simulink model "CLVF"  (R2020a)
settings: Solver=FixedStepAuto  StartTime=0.0  StopTime=tsim  FixedStep=baseRate  RelTol=1e-3  EnableMultiTasking=on
values from neighbouring files (symbols this model uses):
  a = sqrt(sum(aTimesOVec.^2))    [Run_Initializer.m]    (also in a_max_CLVF2D.m = params(4))
  a_max = 0.4/BLACKMass    [Run_Initializer.m]
  a_prime = newParams(2)    [Run_Initializer.m]    (also in a_max_LVF.m = params(2))
  acceptableRadius = 0.05    [Run_Initializer.m]
  b = newParams(3)    [Run_Initializer.m]    (also in a_max_CLVF2D.m = params(3))
  baseRate = 0.05    [Run_Initializer.m]
  BLACKMass = model_param(3)    [Run_Initializer.m]
  d = [0.16;0.542;0]    [Run_Initializer.m]    (also in a_max_LVF.m = [rotStuff(3);rotStuff(4);rotStuff(5)])
  drop_states_BLACK = rC_I0    [Run_Initializer.m]
  drop_states_BLUE = [ xLength/2+0.9; yLength/2+0.5; 0]    [Run_Initializer.m]
  drop_states_RED = rT_I0    [Run_Initializer.m]
  F_thrusters_BLACK = 0.25.*ones(8,1)    [Run_Initializer.m]
  F_thrusters_BLUE = 0.25.*ones(8,1)    [Run_Initializer.m]
  F_thrusters_RED = 0.25.*ones(8,1)    [Run_Initializer.m]
  home_states_BLACK = [ xLength/2+0.4; yLength/2; 0]    [Run_Initializer.m]
  home_states_BLUE = [ xLength/2-0.9; yLength/2+0.5; 0]    [Run_Initializer.m]
  home_states_RED = [ xLength/2-0.4; yLength/2; 0]    [Run_Initializer.m]
  init_states_BLACK = rC_I0    [Run_Initializer.m]
  init_states_BLUE = [ xLength/2+0.9; yLength/2+0.5; 0]    [Run_Initializer.m]
  init_states_RED = rT_I0    [Run_Initializer.m]
  k_v_rel = 2*v_max/a_prime    (= 1)    [Run_Initializer.m]
  ka = newParams(2)    [Run_Initializer.m]    (also in a_max_CLVF2D.m = params(2))
  kc = newParams(1)    [Run_Initializer.m]    (also in a_max_CLVF2D.m = params(1))
  kd = 5.0    (= 5)    [Run_Initializer.m]
  Kd_tb = 0.4    [Run_Initializer.m]
  Kd_tblue = 0.4    [Run_Initializer.m]
  Kd_tr = 0.4    [Run_Initializer.m]
  Kd_xb = 5    [Run_Initializer.m]
  Kd_xblue = 5    [Run_Initializer.m]
  Kd_xr = 5    [Run_Initializer.m]
  Kd_yb = 5    [Run_Initializer.m]
  Kd_yblue = 5    [Run_Initializer.m]
  Kd_yr = 5    [Run_Initializer.m]
  Kp_tb = 0.1    [Run_Initializer.m]
  Kp_tblue = 0.1    [Run_Initializer.m]
  Kp_tr = 0.1    [Run_Initializer.m]
  Kp_xb = 2    [Run_Initializer.m]
  Kp_xblue = 2    [Run_Initializer.m]
  Kp_xr = 2    [Run_Initializer.m]
  Kp_yb = 2    [Run_Initializer.m]
  Kp_yblue = 2    [Run_Initializer.m]
  Kp_yr = 2    [Run_Initializer.m]
  noise_variance_BLACK = 0    [Run_Initializer.m]
  noise_variance_BLUE = 0    [Run_Initializer.m]
  noise_variance_RED = 0    [Run_Initializer.m]
  o_hat_B = aTimesOVec./a    [Run_Initializer.m]
  o_hat_prime = o_prime/sqrt(sum(o_prime.^2))    [Run_Initializer.m]
  Phase0_End = Phase0_Duration    (= 10)    [Run_Initializer.m]
  Phase1_End = Phase0_Duration + Phase1_Duration    (= 15)    [Run_Initializer.m]
  Phase2_End = Phase0_Duration + Phase1_Duration +                                   Phase2_Duration    (= 35)    [Run_Initializer.m]
  Phase3_End = Phase0_Duration + Phase1_Duration +                                   Phase2_Duration + Phase3_Duration    [Run_Initializer.m]
  Phase3_SubPhase1_End = Phase2_End + Phase3_SubPhase1_Duration    (= 40)    [Run_Initializer.m]
  Phase3_SubPhase2_End = Phase2_End + Phase3_SubPhase1_Duration +                                   Phase3_SubPhase2_Duration    (= 45)    [Run_Initializer.m]
  Phase3_SubPhase3_End_BLACK = Phase2_End + Phase3_SubPhase1_Duration +                                   Phase3_SubPhase2_Duration +                                  Phase3_SubPhase3_Duration + Phase3_SubPhase3_and_a_half    (= 51)    [Run_Initializer.m]
  Phase3_SubPhase3_End_RED = Phase2_End + Phase3_SubPhase1_Duration +                                   Phase3_SubPhase2_Duration +                                  Phase3_SubPhase3_Duration    (= 46)    [Run_Initializer.m]
  Phase3_SubPhase4_End = Phase2_End + Phase3_SubPhase1_Duration +                                   Phase3_SubPhase2_Duration +                                  Phase3_SubPhase3_Duration +                                  Phase3_SubPhase4_Duration + Phase3_SubPhase3_and_a_half    [Run_Initializer.m]
  Phase4_End = Phase0_Duration + Phase1_Duration +                                   Phase2_Duration + Phase3_Duration +                                   Phase4_Duration    [Run_Initializer.m]
  Phase5_End = Phase0_Duration + Phase1_Duration +                                   Phase2_Duration + Phase3_Duration +                                   Phase4_Duration + Phase5_Duration    [Run_Initializer.m]
  r_co = r_co_over_a_prime*a_prime    (= 0.16)    [Run_Initializer.m]
  rC_I0 = [0.9*xLength;yLength/2-0.5;pi/2]    [Run_Initializer.m]
  rT_I0 = [yLength/2;yLength/2;possibleStarts(startingRotation)]    [Run_Initializer.m]
  serverRate = 0.1    [Run_Initializer.m]
  sys_BLACK = c2d(sys_BLACK_CONT, baseRate)    [Run_Initializer.m]
  sys_BLACK_ROT = c2d(sys_BLACK_rot_CONT, baseRate)    [Run_Initializer.m]
  sys_RED = c2d(sys_RED_CONT, baseRate)    [Run_Initializer.m]
  sys_RED_ROT = c2d(sys_RED_rot_CONT, baseRate)    [Run_Initializer.m]
  theta_d = 30*d2r    (= 0.523598775598)    [Run_Initializer.m]    (also in a_max_LVF.m = rotStuff(2))
  thruster_dist2CG_BLACK = [83.42;-52.58;55.94;-60.05;54.08;-53.92;77.06;-55.94]    [Run_Initializer.m]
  thruster_dist2CG_BLUE = [83.42;-52.58;55.94;-60.05;54.08;-53.92;77.06;-55.94]    [Run_Initializer.m]
  thruster_dist2CG_RED = [49.92;-78.08;70.46;-63.54;81.08;-50.42;57.44;-75.96]    [Run_Initializer.m]
  w_body = 6.0 * d2r    (= 0.10471975512)    [Run_Initializer.m]
undefined symbols (not defined in the file or in its folder): DiscIntNeverNeededParam, Discrete, Phase3_SubPhase3_End, platformSelection, simMode, Time, WhoAmI
libraries: dspstat3 x18, dspsigops x14, raspberrypiBasiclib x10, embdlinuxlib x8, simulink x8, ctrlSharedLib x4, mspfiltlib x3, dsparch4 x3, dspswit3 x2, MainLibrary x2, sensehatlib x1
(part 8 of 10)

== system CLVF/Gyroscope & Acceleration Algorithms/Change BLUE Behavior/Fix Initial Bias (Accel)/Correct AccelY/Calculate Running Mean ==
  In1 : Inport
  Action Port : ActionPort
  Delay : Delay  DelayLength=1
  Delay1 : Delay
  Delay2 : Delay  DelayLength=4
  Delay3 : Delay  DelayLength=5
  Delay4 : Delay  DelayLength=3
  Mean : dspstat3/Mean  run=off  InputProcessing=Columns as channels (frame based)  reset_popup=None  directionMode=Each column  dimension=1  roiEnable=off  roiType=Rectangles  roiPortion=Entire ROI  roiOutput=Individual statistics for each ROI  roiFlag=off  roundingMode=Floor  overflowMode=off  outputDataTypeStr=Inherit: Same as accumulator  outputMin=[]  outputMax=[]  outputLastDataTypeStr=Inherit: Same as accumulator
  Mux : Mux  Inputs=6
  Out1 : Outport
  wires:
  Delay3/1 -> Mux/6
  Delay2/1 -> Mux/5
  Delay1/1 -> Mux/3
  Delay4/1 -> Mux/4
  Delay/1 -> Mux/2
  In1/1 -> Delay3/1, Delay2/1, Delay4/1, Delay1/1, Delay/1, Mux/1
  Mux/1 -> Mean/1
  Mean/1 -> Out1/1

== system CLVF/Gyroscope & Acceleration Algorithms/Change BLUE Behavior/Fix Initial Bias (Accel)/Correct AccelY/Pass Current Accel ==
  In1 : Inport
  Action Port : ActionPort
  Out1 : Outport
  wires:
  In1/1 -> Out1/1

== system CLVF/Gyroscope & Acceleration Algorithms/Change BLUE Behavior/Fix Initial Bias (Accel)/Correct AccelY/Subsystem ==
  Universal_Time : DataStoreRead  DataStoreName=Univ_Time
  Time : Outport  VectorParamsAs1DForOutWhenUnconnected=off
  wires:
  Universal_Time/1 -> Time/1

== system CLVF/Gyroscope & Acceleration Algorithms/Change BLUE Behavior/Fix Initial Bias (Accel)/Correct AccelZ/Calculate Running Mean ==
  In1 : Inport
  Action Port : ActionPort
  Constant : Constant  Value=9.81
  Delay : Delay  DelayLength=1
  Delay1 : Delay
  Delay2 : Delay  DelayLength=4
  Delay3 : Delay  DelayLength=5
  Delay4 : Delay  DelayLength=3
  Mean : dspstat3/Mean  run=off  InputProcessing=Columns as channels (frame based)  reset_popup=None  directionMode=Each column  dimension=1  roiEnable=off  roiType=Rectangles  roiPortion=Entire ROI  roiOutput=Individual statistics for each ROI  roiFlag=off  roundingMode=Floor  overflowMode=off  outputDataTypeStr=Inherit: Same as accumulator  outputMin=[]  outputMax=[]  outputLastDataTypeStr=Inherit: Same as accumulator
  Mux : Mux  Inputs=6
  Subtract : Sum  Inputs=+-
  Out1 : Outport
  wires:
  Delay3/1 -> Mux/6
  Delay2/1 -> Mux/5
  Delay1/1 -> Mux/3
  Delay4/1 -> Mux/4
  Delay/1 -> Mux/2
  In1/1 -> Delay3/1, Delay2/1, Delay4/1, Delay1/1, Delay/1, Mux/1
  Mux/1 -> Mean/1
  Subtract/1 -> Out1/1
  Mean/1 -> Subtract/1
  Constant/1 -> Subtract/2

== system CLVF/Gyroscope & Acceleration Algorithms/Change BLUE Behavior/Fix Initial Bias (Accel)/Correct AccelZ/Pass Current Accel ==
  In1 : Inport
  Action Port : ActionPort
  Out1 : Outport
  wires:
  In1/1 -> Out1/1

== system CLVF/Gyroscope & Acceleration Algorithms/Change BLUE Behavior/Fix Initial Bias (Accel)/Correct AccelZ/Subsystem ==
  Universal_Time : DataStoreRead  DataStoreName=Univ_Time
  Time : Outport  VectorParamsAs1DForOutWhenUnconnected=off
  wires:
  Universal_Time/1 -> Time/1

== system CLVF/Gyroscope & Acceleration Algorithms/Change RED Behavior/Fix Initial Bias/Correct GyroX/Calculate Running Mean ==
  In1 : Inport
  Action Port : ActionPort
  Delay : Delay  DelayLength=1
  Delay1 : Delay
  Delay2 : Delay  DelayLength=4
  Delay3 : Delay  DelayLength=5
  Delay4 : Delay  DelayLength=3
  Mean : dspstat3/Mean  run=off  InputProcessing=Columns as channels (frame based)  reset_popup=None  directionMode=Each column  dimension=1  roiEnable=off  roiType=Rectangles  roiPortion=Entire ROI  roiOutput=Individual statistics for each ROI  roiFlag=off  roundingMode=Floor  overflowMode=off  outputDataTypeStr=Inherit: Same as accumulator  outputMin=[]  outputMax=[]  outputLastDataTypeStr=Inherit: Same as accumulator
  Mux : Mux  Inputs=6
  Out1 : Outport
  wires:
  Delay3/1 -> Mux/6
  Delay2/1 -> Mux/5
  Delay1/1 -> Mux/3
  Delay4/1 -> Mux/4
  Delay/1 -> Mux/2
  In1/1 -> Delay3/1, Delay2/1, Delay4/1, Delay1/1, Delay/1, Mux/1
  Mux/1 -> Mean/1
  Mean/1 -> Out1/1

== system CLVF/Gyroscope & Acceleration Algorithms/Change RED Behavior/Fix Initial Bias/Correct GyroX/Pass Current Gyro ==
  In1 : Inport
  Action Port : ActionPort
  Out1 : Outport
  wires:
  In1/1 -> Out1/1

== system CLVF/Gyroscope & Acceleration Algorithms/Change RED Behavior/Fix Initial Bias/Correct GyroX/Subsystem ==
  Universal_Time : DataStoreRead  DataStoreName=Univ_Time
  Time : Outport  VectorParamsAs1DForOutWhenUnconnected=off
  wires:
  Universal_Time/1 -> Time/1

== system CLVF/Gyroscope & Acceleration Algorithms/Change RED Behavior/Fix Initial Bias/Correct GyroY/Calculate Running Mean ==
  In1 : Inport
  Action Port : ActionPort
  Delay : Delay  DelayLength=1
  Delay1 : Delay
  Delay2 : Delay  DelayLength=4
  Delay3 : Delay  DelayLength=5
  Delay4 : Delay  DelayLength=3
  Mean : dspstat3/Mean  run=off  InputProcessing=Columns as channels (frame based)  reset_popup=None  directionMode=Each column  dimension=1  roiEnable=off  roiType=Rectangles  roiPortion=Entire ROI  roiOutput=Individual statistics for each ROI  roiFlag=off  roundingMode=Floor  overflowMode=off  outputDataTypeStr=Inherit: Same as accumulator  outputMin=[]  outputMax=[]  outputLastDataTypeStr=Inherit: Same as accumulator
  Mux : Mux  Inputs=6
  Out1 : Outport
  wires:
  Delay3/1 -> Mux/6
  Delay2/1 -> Mux/5
  Delay1/1 -> Mux/3
  Delay4/1 -> Mux/4
  Delay/1 -> Mux/2
  In1/1 -> Delay3/1, Delay2/1, Delay4/1, Delay1/1, Delay/1, Mux/1
  Mux/1 -> Mean/1
  Mean/1 -> Out1/1

== system CLVF/Gyroscope & Acceleration Algorithms/Change RED Behavior/Fix Initial Bias/Correct GyroY/Pass Current Gyro ==
  In1 : Inport
  Action Port : ActionPort
  Out1 : Outport
  wires:
  In1/1 -> Out1/1

== system CLVF/Gyroscope & Acceleration Algorithms/Change RED Behavior/Fix Initial Bias/Correct GyroY/Subsystem ==
  Universal_Time : DataStoreRead  DataStoreName=Univ_Time
  Time : Outport  VectorParamsAs1DForOutWhenUnconnected=off
  wires:
  Universal_Time/1 -> Time/1

== system CLVF/Gyroscope & Acceleration Algorithms/Change RED Behavior/Fix Initial Bias/Correct GyroZ/Calculate Running Mean ==
  In1 : Inport
  Action Port : ActionPort
  Delay : Delay  DelayLength=1
  Delay1 : Delay
  Delay2 : Delay  DelayLength=4
  Delay3 : Delay  DelayLength=5
  Delay4 : Delay  DelayLength=3
  Mean : dspstat3/Mean  run=off  InputProcessing=Columns as channels (frame based)  reset_popup=None  directionMode=Each column  dimension=1  roiEnable=off  roiType=Rectangles  roiPortion=Entire ROI  roiOutput=Individual statistics for each ROI  roiFlag=off  roundingMode=Floor  overflowMode=off  outputDataTypeStr=Inherit: Same as accumulator  outputMin=[]  outputMax=[]  outputLastDataTypeStr=Inherit: Same as accumulator
  Mux : Mux  Inputs=6
  Out1 : Outport
  wires:
  Delay3/1 -> Mux/6
  Delay2/1 -> Mux/5
  Delay1/1 -> Mux/3
  Delay4/1 -> Mux/4
  Delay/1 -> Mux/2
  In1/1 -> Delay3/1, Delay2/1, Delay4/1, Delay1/1, Delay/1, Mux/1
  Mux/1 -> Mean/1
  Mean/1 -> Out1/1

== system CLVF/Gyroscope & Acceleration Algorithms/Change RED Behavior/Fix Initial Bias/Correct GyroZ/Pass Current Gyro ==
  In1 : Inport
  Action Port : ActionPort
  Out1 : Outport
  wires:
  In1/1 -> Out1/1

== system CLVF/Gyroscope & Acceleration Algorithms/Change RED Behavior/Fix Initial Bias/Correct GyroZ/Subsystem ==
  Universal_Time : DataStoreRead  DataStoreName=Univ_Time
  Time : Outport  VectorParamsAs1DForOutWhenUnconnected=off
  wires:
  Universal_Time/1 -> Time/1

== system CLVF/Gyroscope & Acceleration Algorithms/Change RED Behavior/Fix Initial Bias (Accel)/Correct AccelX/Calculate Running Mean ==
  In1 : Inport
  Action Port : ActionPort
  Delay : Delay  DelayLength=1
  Delay1 : Delay
  Delay2 : Delay  DelayLength=4
  Delay3 : Delay  DelayLength=5
  Delay4 : Delay  DelayLength=3
  Mean : dspstat3/Mean  run=off  InputProcessing=Columns as channels (frame based)  reset_popup=None  directionMode=Each column  dimension=1  roiEnable=off  roiType=Rectangles  roiPortion=Entire ROI  roiOutput=Individual statistics for each ROI  roiFlag=off  roundingMode=Floor  overflowMode=off  outputDataTypeStr=Inherit: Same as accumulator  outputMin=[]  outputMax=[]  outputLastDataTypeStr=Inherit: Same as accumulator
  Mux : Mux  Inputs=6
  Out1 : Outport
  wires:
  Delay3/1 -> Mux/6
  Delay2/1 -> Mux/5
  Delay1/1 -> Mux/3
  Delay4/1 -> Mux/4
  Delay/1 -> Mux/2
  In1/1 -> Delay3/1, Delay2/1, Delay4/1, Delay1/1, Delay/1, Mux/1
  Mux/1 -> Mean/1
  Mean/1 -> Out1/1

== system CLVF/Gyroscope & Acceleration Algorithms/Change RED Behavior/Fix Initial Bias (Accel)/Correct AccelX/Pass Current Accel ==
  In1 : Inport
  Action Port : ActionPort
  Out1 : Outport
  wires:
  In1/1 -> Out1/1

== system CLVF/Gyroscope & Acceleration Algorithms/Change RED Behavior/Fix Initial Bias (Accel)/Correct AccelX/Subsystem ==
  Universal_Time : DataStoreRead  DataStoreName=Univ_Time
  Time : Outport  VectorParamsAs1DForOutWhenUnconnected=off
  wires:
  Universal_Time/1 -> Time/1

== system CLVF/Gyroscope & Acceleration Algorithms/Change RED Behavior/Fix Initial Bias (Accel)/Correct AccelY/Calculate Running Mean ==
  In1 : Inport
  Action Port : ActionPort
  Delay : Delay  DelayLength=1
  Delay1 : Delay
  Delay2 : Delay  DelayLength=4
  Delay3 : Delay  DelayLength=5
  Delay4 : Delay  DelayLength=3
  Mean : dspstat3/Mean  run=off  InputProcessing=Columns as channels (frame based)  reset_popup=None  directionMode=Each column  dimension=1  roiEnable=off  roiType=Rectangles  roiPortion=Entire ROI  roiOutput=Individual statistics for each ROI  roiFlag=off  roundingMode=Floor  overflowMode=off  outputDataTypeStr=Inherit: Same as accumulator  outputMin=[]  outputMax=[]  outputLastDataTypeStr=Inherit: Same as accumulator
  Mux : Mux  Inputs=6
  Out1 : Outport
  wires:
  Delay3/1 -> Mux/6
  Delay2/1 -> Mux/5
  Delay1/1 -> Mux/3
  Delay4/1 -> Mux/4
  Delay/1 -> Mux/2
  In1/1 -> Delay3/1, Delay2/1, Delay4/1, Delay1/1, Delay/1, Mux/1
  Mux/1 -> Mean/1
  Mean/1 -> Out1/1

== system CLVF/Gyroscope & Acceleration Algorithms/Change RED Behavior/Fix Initial Bias (Accel)/Correct AccelY/Pass Current Accel ==
  In1 : Inport
  Action Port : ActionPort
  Out1 : Outport
  wires:
  In1/1 -> Out1/1

== system CLVF/Gyroscope & Acceleration Algorithms/Change RED Behavior/Fix Initial Bias (Accel)/Correct AccelY/Subsystem ==
  Universal_Time : DataStoreRead  DataStoreName=Univ_Time
  Time : Outport  VectorParamsAs1DForOutWhenUnconnected=off
  wires:
  Universal_Time/1 -> Time/1

== system CLVF/Gyroscope & Acceleration Algorithms/Change RED Behavior/Fix Initial Bias (Accel)/Correct AccelZ/Calculate Running Mean ==
  In1 : Inport
  Action Port : ActionPort
  Constant : Constant  Value=9.81
  Delay : Delay  DelayLength=1
  Delay1 : Delay
  Delay2 : Delay  DelayLength=4
  Delay3 : Delay  DelayLength=5
  Delay4 : Delay  DelayLength=3
  Mean : dspstat3/Mean  run=off  InputProcessing=Columns as channels (frame based)  reset_popup=None  directionMode=Each column  dimension=1  roiEnable=off  roiType=Rectangles  roiPortion=Entire ROI  roiOutput=Individual statistics for each ROI  roiFlag=off  roundingMode=Floor  overflowMode=off  outputDataTypeStr=Inherit: Same as accumulator  outputMin=[]  outputMax=[]  outputLastDataTypeStr=Inherit: Same as accumulator
  Mux : Mux  Inputs=6
  Subtract : Sum  Inputs=+-
  Out1 : Outport
  wires:
  Delay3/1 -> Mux/6
  Delay2/1 -> Mux/5
  Delay1/1 -> Mux/3
  Delay4/1 -> Mux/4
  Delay/1 -> Mux/2
  In1/1 -> Delay3/1, Delay2/1, Delay4/1, Delay1/1, Delay/1, Mux/1
  Mux/1 -> Mean/1
  Subtract/1 -> Out1/1
  Mean/1 -> Subtract/1
  Constant/1 -> Subtract/2

== system CLVF/Gyroscope & Acceleration Algorithms/Change RED Behavior/Fix Initial Bias (Accel)/Correct AccelZ/Pass Current Accel ==
  In1 : Inport
  Action Port : ActionPort
  Out1 : Outport
  wires:
  In1/1 -> Out1/1

== system CLVF/Gyroscope & Acceleration Algorithms/Change RED Behavior/Fix Initial Bias (Accel)/Correct AccelZ/Subsystem ==
  Universal_Time : DataStoreRead  DataStoreName=Univ_Time
  Time : Outport  VectorParamsAs1DForOutWhenUnconnected=off
  wires:
  Universal_Time/1 -> Time/1

== system CLVF/Phase #2: Move to Initial Position/Change BLACK Behavior/Custom Discrete PD (Attitude)/x_dot -> x1/Hold this value ==
  In1 : Inport
  Action Port : ActionPort  ActionPortLabel=if(u1 ~= 0)
  Out1 : Outport  VectorParamsAs1DForOutWhenUnconnected=off
  wires:
  In1/1 -> Out1/1

== system CLVF/Phase #2: Move to Initial Position/Change BLACK Behavior/Custom Discrete PD (X-Position)/x_dot -> x1/Hold this value ==
  In1 : Inport
  Action Port : ActionPort  ActionPortLabel=if(u1 ~= 0)
  Out1 : Outport  VectorParamsAs1DForOutWhenUnconnected=off
  wires:
  In1/1 -> Out1/1

== system CLVF/Phase #2: Move to Initial Position/Change BLACK Behavior/Custom Discrete PD (Y-Position)/x_dot -> x1/Hold this value ==
  In1 : Inport
  Action Port : ActionPort  ActionPortLabel=if(u1 ~= 0)
  Out1 : Outport  VectorParamsAs1DForOutWhenUnconnected=off
  wires:
  In1/1 -> Out1/1

== system CLVF/Phase #2: Move to Initial Position/Change BLUE Behavior/Custom Discrete PD (Attitude)/x_dot -> x1/Hold this value ==
  In1 : Inport
  Action Port : ActionPort  ActionPortLabel=if(u1 ~= 0)
  Out1 : Outport  VectorParamsAs1DForOutWhenUnconnected=off
  wires:
  In1/1 -> Out1/1

== system CLVF/Phase #2: Move to Initial Position/Change BLUE Behavior/Custom Discrete PD (X-Position)/x_dot -> x1/Hold this value ==
  In1 : Inport
  Action Port : ActionPort  ActionPortLabel=if(u1 ~= 0)
  Out1 : Outport  VectorParamsAs1DForOutWhenUnconnected=off
  wires:
  In1/1 -> Out1/1

== system CLVF/Phase #2: Move to Initial Position/Change BLUE Behavior/Custom Discrete PD (Y-Position)/x_dot -> x1/Hold this value ==
  In1 : Inport
  Action Port : ActionPort  ActionPortLabel=if(u1 ~= 0)
  Out1 : Outport  VectorParamsAs1DForOutWhenUnconnected=off
  wires:
  In1/1 -> Out1/1

== system CLVF/Phase #2: Move to Initial Position/Change RED Behavior/Custom Discrete PD (Attitude)/x_dot -> x1/Hold this value ==
  In1 : Inport
  Action Port : ActionPort  ActionPortLabel=if(u1 ~= 0)
  Out1 : Outport  VectorParamsAs1DForOutWhenUnconnected=off
  wires:
  In1/1 -> Out1/1

== system CLVF/Phase #2: Move to Initial Position/Change RED Behavior/Custom Discrete PD (X-Position)/x_dot -> x1/Hold this value ==
  In1 : Inport
  Action Port : ActionPort  ActionPortLabel=if(u1 ~= 0)
  Out1 : Outport  VectorParamsAs1DForOutWhenUnconnected=off
  wires:
  In1/1 -> Out1/1

== system CLVF/Phase #2: Move to Initial Position/Change RED Behavior/Custom Discrete PD (Y-Position)/x_dot -> x1/Hold this value ==
  In1 : Inport
  Action Port : ActionPort  ActionPortLabel=if(u1 ~= 0)
  Out1 : Outport  VectorParamsAs1DForOutWhenUnconnected=off
  wires:
  In1/1 -> Out1/1

== system CLVF/Phase #3: Experiment/Change BLACK Behavior/Sub-Phase #1/Custom Discrete PD (Attitude)/x_dot -> x1 ==
  note: dy/dt ~= (y2-y1)/deltaT
  y(t) : Inport
  Delay1 : Delay  DelayLength=1  InitialConditionSource=Input port
      settings: InputPortMap=u0,p4
  Hold this value : Subsystem  TreatAsAtomicUnit=on
  Sum6 : Sum  Inputs=-+|
  divide by delta T : Gain  Gain=1/serverRate
  "if we went through a \"step\"" : If  IfExpression=u1 ~= 0  ShowElse=off
  dy(t)/dt : Outport  VectorParamsAs1DForOutWhenUnconnected=off
  wires:
  divide by delta T/1 -> dy(t)/dt/1
  Delay1/1 -> Sum6/1
  "if we went through a \"step\""/1 -> Hold this value/Action
  Hold this value/1(Out1) -> divide by delta T/1
  Sum6/1 -> "if we went through a \"step\""/1, Hold this value/1(In1)
  y(t)/1 -> Sum6/2, Delay1/2, Delay1/1

== system CLVF/Phase #3: Experiment/Change BLACK Behavior/Sub-Phase #1/Custom Discrete PD (X-Position)/x_dot -> x1 ==
  note: dy/dt ~= (y2-y1)/deltaT
  y(t) : Inport
  Delay1 : Delay  DelayLength=1  InitialConditionSource=Input port
      settings: InputPortMap=u0,p4
  Hold this value : Subsystem  TreatAsAtomicUnit=on
  Sum6 : Sum  Inputs=-+|
  divide by delta T : Gain  Gain=1/serverRate
  "if we went through a \"step\"" : If  IfExpression=u1 ~= 0  ShowElse=off
  dy(t)/dt : Outport  VectorParamsAs1DForOutWhenUnconnected=off
  wires:
  divide by delta T/1 -> dy(t)/dt/1
  Delay1/1 -> Sum6/1
  "if we went through a \"step\""/1 -> Hold this value/Action
  Hold this value/1(Out1) -> divide by delta T/1
  Sum6/1 -> "if we went through a \"step\""/1, Hold this value/1(In1)
  y(t)/1 -> Sum6/2, Delay1/2, Delay1/1

== system CLVF/Phase #3: Experiment/Change BLACK Behavior/Sub-Phase #1/Custom Discrete PD (Y-Position)/x_dot -> x1 ==
  note: dy/dt ~= (y2-y1)/deltaT
  y(t) : Inport
  Delay1 : Delay  DelayLength=1  InitialConditionSource=Input port
      settings: InputPortMap=u0,p4
  Hold this value : Subsystem  TreatAsAtomicUnit=on
  Sum6 : Sum  Inputs=-+|
  divide by delta T : Gain  Gain=1/serverRate
  "if we went through a \"step\"" : If  IfExpression=u1 ~= 0  ShowElse=off
  dy(t)/dt : Outport  VectorParamsAs1DForOutWhenUnconnected=off
  wires:
  divide by delta T/1 -> dy(t)/dt/1
  Delay1/1 -> Sum6/1
  "if we went through a \"step\""/1 -> Hold this value/Action
  Hold this value/1(Out1) -> divide by delta T/1
  Sum6/1 -> "if we went through a \"step\""/1, Hold this value/1(In1)
  y(t)/1 -> Sum6/2, Delay1/2, Delay1/1

== system CLVF/Phase #3: Experiment/Change BLACK Behavior/Sub-Phase #4/BLACK_RzD/Subsystem ==
  Constant1 : Constant  Value=Phase3_SubPhase3_End  SampleTime=-1
  Subtract : Sum  Inputs=+-
  Universal_Time : DataStoreRead  DataStoreName=Univ_Time
  Time : Outport  VectorParamsAs1DForOutWhenUnconnected=off
  wires:
  Universal_Time/1 -> Subtract/1
  Subtract/1 -> Time/1
  Constant1/1 -> Subtract/2

== system CLVF/Phase #3: Experiment/Change BLACK Behavior/Sub-Phase #4/BLACK_RzD/Wrap1 ==
  unwrapped : Inport
  MATLAB Function : MATLAB Function  TreatAsAtomicUnit=on
  wrapped : Outport  VectorParamsAs1DForOutWhenUnconnected=off
  wires:
  MATLAB Function/1(wrappedAngle) -> wrapped/1
  unwrapped/1 -> MATLAB Function/1(u)

== system CLVF/Phase #3: Experiment/Change BLACK Behavior/Sub-Phase #4/Custom Discrete PD (Attitude)/x_dot -> x1 ==
  note: dy/dt ~= (y2-y1)/deltaT
  y(t) : Inport
  Delay1 : Delay  DelayLength=1  InitialConditionSource=Input port
      settings: InputPortMap=u0,p4
  Hold this value : Subsystem  TreatAsAtomicUnit=on
  Sum6 : Sum  Inputs=-+|
  divide by delta T : Gain  Gain=1/serverRate
  "if we went through a \"step\"" : If  IfExpression=u1 ~= 0  ShowElse=off
  dy(t)/dt : Outport  VectorParamsAs1DForOutWhenUnconnected=off
  wires:
  divide by delta T/1 -> dy(t)/dt/1
  Delay1/1 -> Sum6/1
  "if we went through a \"step\""/1 -> Hold this value/Action
  Hold this value/1(Out1) -> divide by delta T/1
  Sum6/1 -> "if we went through a \"step\""/1, Hold this value/1(In1)
  y(t)/1 -> Sum6/2, Delay1/2, Delay1/1

== system CLVF/Phase #3: Experiment/Change BLACK Behavior/Sub-Phase #4/Lyapunov GNC/CLVF Approach ==
  rC_T : Inport
  vC_I : Inport  Port=2
  vT_I : Inport  Port=3
  theta_T : Inport  Port=4
  theta_dot_T : Inport  Port=5
  Action Port : ActionPort  ActionPortLabel=if(u1 == 0)
  CLVF Guidance : MATLAB Function  TreatAsAtomicUnit=on
  Constant : Constant  Value=[0;0;0]
  Constant1 : Constant  Value=0
  Scope10 : Scope
  Scope8 : Scope
  Scope9 : Scope
  Sum : Sum  Inputs=|+-
  Sum1 : Sum  Inputs=|+-
  Terminator : Terminator
  Vec Derivative : Subsystem
  h : Outport  VectorParamsAs1DForOutWhenUnconnected=off
  a_ff : Outport  Port=2  VectorParamsAs1DForOutWhenUnconnected=off
  r : Outport  Port=3  VectorParamsAs1DForOutWhenUnconnected=off
  alignmentAngle : Outport  Port=4  VectorParamsAs1DForOutWhenUnconnected=off
  wires:
  Sum/1 -> CLVF Guidance/2(vC_T)
  vC_I/1 -> Sum/1
  vT_I/1 -> CLVF Guidance/3(vT_I), Sum/2
  CLVF Guidance/1(h) -> h/1, Vec Derivative/1(In1)
  Constant1/1 -> CLVF Guidance/7(theta_ddot)
  Constant/1 -> CLVF Guidance/4(aT_I)
  CLVF Guidance/2(a_ff) -> a_ff/1, Sum1/2, Scope9/1
  rC_T/1 -> CLVF Guidance/1(rC_T)
  theta_T/1 -> CLVF Guidance/5(theta)
  theta_dot_T/1 -> CLVF Guidance/6(theta_dot)
  Vec Derivative/1(Out1) -> Sum1/1, Scope8/1
  Sum1/1 -> Scope10/1
  CLVF Guidance/3(r) -> r/1
  CLVF Guidance/4(alignmentAngle) -> alignmentAngle/1
  CLVF Guidance/5(o_hat) -> Terminator/1

== system CLVF/Phase #3: Experiment/Change BLACK Behavior/Sub-Phase #4/Lyapunov GNC/Lyapunov ==
  note: LVF Docking Guidance
  note: INPUTS
  rC_T : Inport
  vC_I : Inport  Port=2
  vT_I : Inport  Port=3
  theta : Inport  Port=4
  theta_dot : Inport  Port=5
  Action Port : ActionPort  ActionPortLabel=else
  Body-Fixed Guidance : MATLAB Function  TreatAsAtomicUnit=on
  Constant : Constant  Value=0
  Scope10 : Scope
  Scope8 : Scope
  Scope9 : Scope
  Sum : Sum  Inputs=|+-
  Sum1 : Sum  Inputs=|+-
  Vec Derivative : Subsystem
  h : Outport
  a_ff : Outport  Port=2
  r : Outport  Port=3
  newTheta : Outport  Port=4
  o_hat_docking : Outport  Port=5  VectorParamsAs1DForOutWhenUnconnected=off
  wires:
  rC_T/1 -> [rC_T]
  vC_I/1 -> [vC_I]
  theta/1 -> [theta]
  theta_dot/1 -> [theta_dot]
  [rC_T] -> Body-Fixed Guidance/1(rC_T)
  [theta_dot] -> Body-Fixed Guidance/3(theta_dot)
  [theta] -> Body-Fixed Guidance/2(theta)
  Constant/1 -> Body-Fixed Guidance/4(theta_ddot)
  vT_I/1 -> [vT_I]
  [vT_I] -> Body-Fixed Guidance/5(vT_I)
  Body-Fixed Guidance/3(r) -> r/1
  Body-Fixed Guidance/4(newTheta) -> newTheta/1
  [vC_I] -> Sum/1
  [vT_I] -> Sum/2
  Sum/1 -> [vC_T]
  [vC_T] -> Body-Fixed Guidance/6(vC_T)
  Body-Fixed Guidance/5(o_hat) -> o_hat_docking/1
  Vec Derivative/1(Out1) -> Sum1/1, Scope8/1
  Body-Fixed Guidance/2(acc_ff) -> Sum1/2, Scope9/1, a_ff/1
  Body-Fixed Guidance/1(hC_T) -> Vec Derivative/1(In1), h/1
  Sum1/1 -> Scope10/1

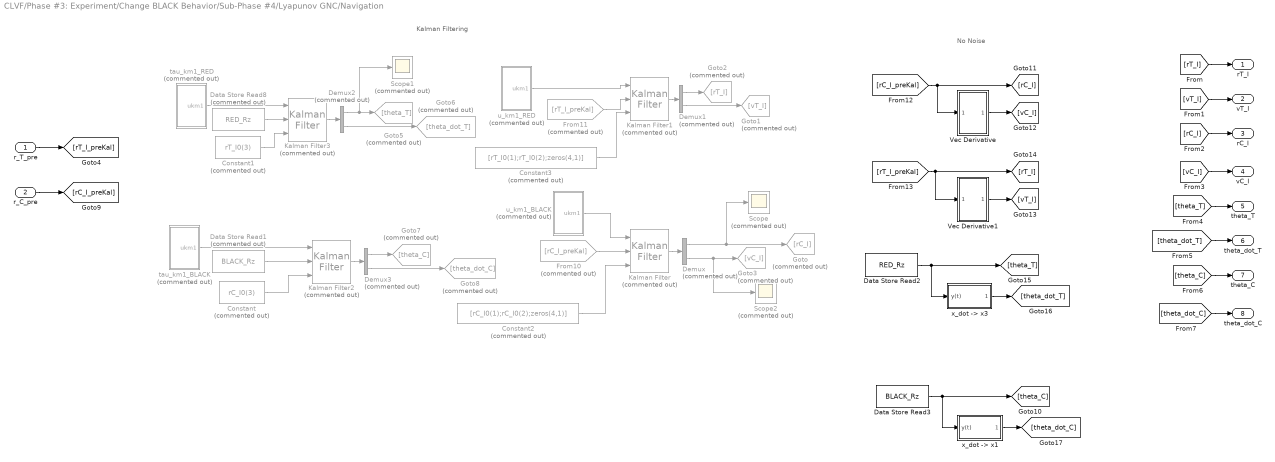
== system CLVF/Phase #3: Experiment/Change BLACK Behavior/Sub-Phase #4/Lyapunov GNC/Navigation ==
  note: Kalman Filtering
  note: No Noise
  r_T_pre : Inport
  r_C_pre : Inport  Port=2
  Constant : Constant  Commented=on  Value=rC_I0(3)
  Constant1 : Constant  Commented=on  Value=rT_I0(3)
  Constant2 : Constant  Commented=on  Value=[rC_I0(1);rC_I0(2);zeros(4,1)]
  Constant3 : Constant  Commented=on  Value=[rT_I0(1);rT_I0(2);zeros(4,1)]
  Data Store Read1 : DataStoreRead  Commented=on  DataStoreName=BLACK_Rz
  Data Store Read2 : DataStoreRead  DataStoreName=RED_Rz
  Data Store Read3 : DataStoreRead  DataStoreName=BLACK_Rz
  Data Store Read8 : DataStoreRead  Commented=on  DataStoreName=RED_Rz
  Demux{,1..3} (4 alike) : Demux  Commented=on  Outputs=2
  From10 : From  Commented=on  GotoTag=rC_I_preKal
  From11 : From  Commented=on  GotoTag=rT_I_preKal
  Goto : Goto  Commented=on  GotoTag=rC_I
  Goto1 : Goto  Commented=on  GotoTag=vT_I
  Goto2 : Goto  Commented=on  GotoTag=rT_I
  Goto3 : Goto  Commented=on  GotoTag=vC_I
  Goto5 : Goto  Commented=on  GotoTag=theta_T
  Goto6 : Goto  Commented=on  GotoTag=theta_dot_T
  Goto7 : Goto  Commented=on  GotoTag=theta_C
  Goto8 : Goto  Commented=on  GotoTag=theta_dot_C
  Kalman Filter : ctrlSharedLib/Kalman Filter  Commented=on  TimeDomain=Discrete-Time  UseCurrentEstimator=on  ModelSource=Individual A, B, C, D matrices  ModelSourceVariable=ss(0.95,1,1,0,1)  A=sys_BLACK.A  B=sys_BLACK.B  C=sys_BLACK.C  D=sys_BLACK.D  NumberOfStates=1  NumberOfInputs=1  NumberOfOutputs=1  InitialEstimateSource=Input port  X0=0  P0=10  UseK=off  UseGH=off  NumberOfProcessNoiseInputs=1  G=1  TimeInvariantG=on  H=0  TimeInvariantH=on  Q=0.01  TimeInvariantQ=on  R=1  TimeInvariantR=on  N=0  TimeInvariantN=on  AddInputPort=on  AddEnablePort=off  OutputEstimatedY=off  OutputP=off  Ts=-1
      settings: SourceProductBaseCode=CT
  Kalman Filter1 : ctrlSharedLib/Kalman Filter  Commented=on  TimeDomain=Discrete-Time  UseCurrentEstimator=on  ModelSource=Individual A, B, C, D matrices  ModelSourceVariable=ss(0.95,1,1,0,1)  A=sys_RED.A  B=sys_RED.B  C=sys_RED.C  D=sys_RED.D  NumberOfStates=1  NumberOfInputs=1  NumberOfOutputs=1  InitialEstimateSource=Input port  X0=0  P0=10  UseK=off  UseGH=off  NumberOfProcessNoiseInputs=1  G=1  TimeInvariantG=on  H=0  TimeInvariantH=on  Q=0.01  TimeInvariantQ=on  R=1  TimeInvariantR=on  N=0  TimeInvariantN=on  AddInputPort=on  AddEnablePort=off  OutputEstimatedY=off  OutputP=off  Ts=-1
      settings: SourceProductBaseCode=CT
  Kalman Filter2 : ctrlSharedLib/Kalman Filter  Commented=on  TimeDomain=Discrete-Time  UseCurrentEstimator=on  ModelSource=Individual A, B, C, D matrices  ModelSourceVariable=ss(0.95,1,1,0,1)  A=sys_BLACK_ROT.A  B=sys_BLACK_ROT.B  C=sys_BLACK_ROT.C  D=sys_BLACK_ROT.D  NumberOfStates=1  NumberOfInputs=1  NumberOfOutputs=1  InitialEstimateSource=Input port  X0=0  P0=10  UseK=off  UseGH=off  NumberOfProcessNoiseInputs=1  G=1  TimeInvariantG=on  H=0  TimeInvariantH=on  Q=0.01  TimeInvariantQ=on  R=1  TimeInvariantR=on  N=0  TimeInvariantN=on  AddInputPort=on  AddEnablePort=off  OutputEstimatedY=off  OutputP=off  Ts=-1
      settings: SourceProductBaseCode=CT
  Kalman Filter3 : ctrlSharedLib/Kalman Filter  Commented=on  TimeDomain=Discrete-Time  UseCurrentEstimator=on  ModelSource=Individual A, B, C, D matrices  ModelSourceVariable=ss(0.95,1,1,0,1)  A=sys_RED_ROT.A  B=sys_RED_ROT.B  C=sys_RED_ROT.C  D=sys_RED_ROT.D  NumberOfStates=1  NumberOfInputs=1  NumberOfOutputs=1  InitialEstimateSource=Input port  X0=0  P0=10  UseK=off  UseGH=off  NumberOfProcessNoiseInputs=1  G=1  TimeInvariantG=on  H=0  TimeInvariantH=on  Q=0.01  TimeInvariantQ=on  R=1  TimeInvariantR=on  N=0  TimeInvariantN=on  AddInputPort=on  AddEnablePort=off  OutputEstimatedY=off  OutputP=off  Ts=-1
      settings: SourceProductBaseCode=CT
  Scope : Scope  Commented=on
  Scope1 : Scope  Commented=on
  Scope2 : Scope  Commented=on
  Vec Derivative : Subsystem
  Vec Derivative1 : Subsystem
  tau_km1_BLACK : Subsystem  Commented=on
  tau_km1_RED : Subsystem  Commented=on
  u_km1_BLACK : Subsystem  Commented=on
  u_km1_RED : Subsystem  Commented=on
  "x_dot -> x1" : Subsystem
  "x_dot -> x3" : Subsystem
  rT_I : Outport  VectorParamsAs1DForOutWhenUnconnected=off
  vT_I : Outport  Port=2  VectorParamsAs1DForOutWhenUnconnected=off
  rC_I : Outport  Port=3  VectorParamsAs1DForOutWhenUnconnected=off
  vC_I : Outport  Port=4  VectorParamsAs1DForOutWhenUnconnected=off
  theta_T : Outport  Port=5  VectorParamsAs1DForOutWhenUnconnected=off
  theta_dot_T : Outport  Port=6  VectorParamsAs1DForOutWhenUnconnected=off
  theta_C : Outport  Port=7  VectorParamsAs1DForOutWhenUnconnected=off
  theta_dot_C : Outport  Port=8  VectorParamsAs1DForOutWhenUnconnected=off
  wires:
  Kalman Filter3/1 -> Demux2/1
  From11/1 -> Kalman Filter1/2
  From10/1 -> Kalman Filter/2
  [rT_I_preKal] -> Vec Derivative1/1(In1), [rT_I]
  Data Store Read1/1 -> Kalman Filter2/2
  u_km1_RED/1(ukm1) -> Kalman Filter1/1
  Demux/1 -> Scope/1, Goto/1
  tau_km1_RED/1(ukm1) -> Kalman Filter3/1
  Data Store Read8/1 -> Kalman Filter3/2
  [rC_I_preKal] -> Vec Derivative/1(In1), [rC_I]
  Data Store Read2/1 -> "x_dot -> x3"/1(y(t)), [theta_T]
  Vec Derivative1/1(Out1) -> [vT_I]
  Demux/2 -> Scope2/1, Goto3/1
  Kalman Filter/1 -> Demux/1
  tau_km1_BLACK/1(ukm1) -> Kalman Filter2/1
  Vec Derivative/1(Out1) -> [vC_I]
  "x_dot -> x3"/1(dy(t)/dt) -> [theta_dot_T]
  u_km1_BLACK/1(ukm1) -> Kalman Filter/1
  Kalman Filter1/1 -> Demux1/1
  Demux1/2 -> Goto1/1
  Demux1/1 -> Goto2/1
  Kalman Filter2/1 -> Demux3/1
  Demux3/1 -> Goto7/1
  Demux3/2 -> Goto8/1
  Demux2/1 -> Scope1/1, Goto5/1
  Demux2/2 -> Goto6/1
  [rT_I] -> rT_I/1
  [vT_I] -> vT_I/1
  [rC_I] -> rC_I/1
  [vC_I] -> vC_I/1
  [theta_T] -> theta_T/1
  [theta_dot_T] -> theta_dot_T/1
  [theta_C] -> theta_C/1
  [theta_dot_C] -> theta_dot_C/1
  r_T_pre/1 -> [rT_I_preKal]
  r_C_pre/1 -> [rC_I_preKal]
  Constant/1 -> Kalman Filter2/3
  Constant1/1 -> Kalman Filter3/3
  Constant2/1 -> Kalman Filter/3
  Constant3/1 -> Kalman Filter1/3
  "x_dot -> x1"/1(dy(t)/dt) -> [theta_dot_C]
  Data Store Read3/1 -> "x_dot -> x1"/1(y(t)), [theta_C]

== system CLVF/Phase #3: Experiment/Change BLACK Behavior/Sub-Phase #4/Lyapunov GNC/SWITCH ==
  rC_T : Inport
  theta : Inport  Port=2
  Delay : Delay  DelayLength=1  InitialCondition=0
  Sample and Hold : dspsigops/Sample and Hold  trig=Rising edge  initCond=0  latchinput=off
  inDesiredRadius : MATLAB Function  TreatAsAtomicUnit=on
  sufficientTime : MATLAB Function  TreatAsAtomicUnit=on
  oneOrZero : Outport
  wires:
  rC_T/1 -> inDesiredRadius/1(rC_T)
  theta/1 -> inDesiredRadius/2(theta)
  Delay/1 -> inDesiredRadius/3(currentCnt)
  inDesiredRadius/1(newCnt) -> sufficientTime/1(cnt), Delay/1
  Sample and Hold/1 -> oneOrZero/1
  sufficientTime/1(oneOrZero) -> Sample and Hold/Trigger, Sample and Hold/1

== system CLVF/Phase #3: Experiment/Change BLUE Behavior/Sub-Phase #1/Custom Discrete PD (Attitude)/x_dot -> x1 ==
  note: dy/dt ~= (y2-y1)/deltaT
  y(t) : Inport
  Delay1 : Delay  DelayLength=1  InitialConditionSource=Input port
      settings: InputPortMap=u0,p4
  Hold this value : Subsystem  TreatAsAtomicUnit=on
  Sum6 : Sum  Inputs=-+|
  divide by delta T : Gain  Gain=1/serverRate
  "if we went through a \"step\"" : If  IfExpression=u1 ~= 0  ShowElse=off
  dy(t)/dt : Outport  VectorParamsAs1DForOutWhenUnconnected=off
  wires:
  divide by delta T/1 -> dy(t)/dt/1
  Delay1/1 -> Sum6/1
  "if we went through a \"step\""/1 -> Hold this value/Action
  Hold this value/1(Out1) -> divide by delta T/1
  Sum6/1 -> "if we went through a \"step\""/1, Hold this value/1(In1)
  y(t)/1 -> Sum6/2, Delay1/2, Delay1/1

== system CLVF/Phase #3: Experiment/Change BLUE Behavior/Sub-Phase #1/Custom Discrete PD (X-Position)/x_dot -> x1 ==
  note: dy/dt ~= (y2-y1)/deltaT
  y(t) : Inport
  Delay1 : Delay  DelayLength=1  InitialConditionSource=Input port
      settings: InputPortMap=u0,p4
  Hold this value : Subsystem  TreatAsAtomicUnit=on
  Sum6 : Sum  Inputs=-+|
  divide by delta T : Gain  Gain=1/serverRate
  "if we went through a \"step\"" : If  IfExpression=u1 ~= 0  ShowElse=off
  dy(t)/dt : Outport  VectorParamsAs1DForOutWhenUnconnected=off
  wires:
  divide by delta T/1 -> dy(t)/dt/1
  Delay1/1 -> Sum6/1
  "if we went through a \"step\""/1 -> Hold this value/Action
  Hold this value/1(Out1) -> divide by delta T/1
  Sum6/1 -> "if we went through a \"step\""/1, Hold this value/1(In1)
  y(t)/1 -> Sum6/2, Delay1/2, Delay1/1

== system CLVF/Phase #3: Experiment/Change BLUE Behavior/Sub-Phase #1/Custom Discrete PD (Y-Position)/x_dot -> x1 ==
  note: dy/dt ~= (y2-y1)/deltaT
  y(t) : Inport
  Delay1 : Delay  DelayLength=1  InitialConditionSource=Input port
      settings: InputPortMap=u0,p4
  Hold this value : Subsystem  TreatAsAtomicUnit=on
  Sum6 : Sum  Inputs=-+|
  divide by delta T : Gain  Gain=1/serverRate
  "if we went through a \"step\"" : If  IfExpression=u1 ~= 0  ShowElse=off
  dy(t)/dt : Outport  VectorParamsAs1DForOutWhenUnconnected=off
  wires:
  divide by delta T/1 -> dy(t)/dt/1
  Delay1/1 -> Sum6/1
  "if we went through a \"step\""/1 -> Hold this value/Action
  Hold this value/1(Out1) -> divide by delta T/1
  Sum6/1 -> "if we went through a \"step\""/1, Hold this value/1(In1)
  y(t)/1 -> Sum6/2, Delay1/2, Delay1/1

== system CLVF/Phase #3: Experiment/Change BLUE Behavior/Sub-Phase #4/Custom Discrete PD (Attitude)/x_dot -> x1 ==
  note: dy/dt ~= (y2-y1)/deltaT
  y(t) : Inport
  Delay1 : Delay  DelayLength=1  InitialConditionSource=Input port
      settings: InputPortMap=u0,p4
  Hold this value : Subsystem  TreatAsAtomicUnit=on
  Sum6 : Sum  Inputs=-+|
  divide by delta T : Gain  Gain=1/serverRate
  "if we went through a \"step\"" : If  IfExpression=u1 ~= 0  ShowElse=off
  dy(t)/dt : Outport  VectorParamsAs1DForOutWhenUnconnected=off
  wires:
  divide by delta T/1 -> dy(t)/dt/1
  Delay1/1 -> Sum6/1
  "if we went through a \"step\""/1 -> Hold this value/Action
  Hold this value/1(Out1) -> divide by delta T/1
  Sum6/1 -> "if we went through a \"step\""/1, Hold this value/1(In1)
  y(t)/1 -> Sum6/2, Delay1/2, Delay1/1

== system CLVF/Phase #3: Experiment/Change BLUE Behavior/Sub-Phase #4/Custom Discrete PD (X-Position)/x_dot -> x1 ==
  note: dy/dt ~= (y2-y1)/deltaT
  y(t) : Inport
  Delay1 : Delay  DelayLength=1  InitialConditionSource=Input port
      settings: InputPortMap=u0,p4
  Hold this value : Subsystem  TreatAsAtomicUnit=on
  Sum6 : Sum  Inputs=-+|
  divide by delta T : Gain  Gain=1/serverRate
  "if we went through a \"step\"" : If  IfExpression=u1 ~= 0  ShowElse=off
  dy(t)/dt : Outport  VectorParamsAs1DForOutWhenUnconnected=off
  wires:
  divide by delta T/1 -> dy(t)/dt/1
  Delay1/1 -> Sum6/1
  "if we went through a \"step\""/1 -> Hold this value/Action
  Hold this value/1(Out1) -> divide by delta T/1
  Sum6/1 -> "if we went through a \"step\""/1, Hold this value/1(In1)
  y(t)/1 -> Sum6/2, Delay1/2, Delay1/1

== system CLVF/Phase #3: Experiment/Change BLUE Behavior/Sub-Phase #4/Custom Discrete PD (Y-Position)/x_dot -> x1 ==
  note: dy/dt ~= (y2-y1)/deltaT
  y(t) : Inport
  Delay1 : Delay  DelayLength=1  InitialConditionSource=Input port
      settings: InputPortMap=u0,p4
  Hold this value : Subsystem  TreatAsAtomicUnit=on
  Sum6 : Sum  Inputs=-+|
  divide by delta T : Gain  Gain=1/serverRate
  "if we went through a \"step\"" : If  IfExpression=u1 ~= 0  ShowElse=off
  dy(t)/dt : Outport  VectorParamsAs1DForOutWhenUnconnected=off
  wires:
  divide by delta T/1 -> dy(t)/dt/1
  Delay1/1 -> Sum6/1
  "if we went through a \"step\""/1 -> Hold this value/Action
  Hold this value/1(Out1) -> divide by delta T/1
  Sum6/1 -> "if we went through a \"step\""/1, Hold this value/1(In1)
  y(t)/1 -> Sum6/2, Delay1/2, Delay1/1

== system CLVF/Phase #3: Experiment/Change RED Behavior/Sub-Phase #1/Custom Discrete PD (Attitude)/x_dot -> x1 ==
  note: dy/dt ~= (y2-y1)/deltaT
  y(t) : Inport
  Delay1 : Delay  DelayLength=1  InitialConditionSource=Input port
      settings: InputPortMap=u0,p4
  Hold this value : Subsystem  TreatAsAtomicUnit=on
  Sum6 : Sum  Inputs=-+|
  divide by delta T : Gain  Gain=1/serverRate
  "if we went through a \"step\"" : If  IfExpression=u1 ~= 0  ShowElse=off
  dy(t)/dt : Outport  VectorParamsAs1DForOutWhenUnconnected=off
  wires:
  divide by delta T/1 -> dy(t)/dt/1
  Delay1/1 -> Sum6/1
  "if we went through a \"step\""/1 -> Hold this value/Action
  Hold this value/1(Out1) -> divide by delta T/1
  Sum6/1 -> "if we went through a \"step\""/1, Hold this value/1(In1)
  y(t)/1 -> Sum6/2, Delay1/2, Delay1/1

== system CLVF/Phase #3: Experiment/Change RED Behavior/Sub-Phase #1/Custom Discrete PD (X-Position)/x_dot -> x1 ==
  note: dy/dt ~= (y2-y1)/deltaT
  y(t) : Inport
  Delay1 : Delay  DelayLength=1  InitialConditionSource=Input port
      settings: InputPortMap=u0,p4
  Hold this value : Subsystem  TreatAsAtomicUnit=on
  Sum6 : Sum  Inputs=-+|
  divide by delta T : Gain  Gain=1/serverRate
  "if we went through a \"step\"" : If  IfExpression=u1 ~= 0  ShowElse=off
  dy(t)/dt : Outport  VectorParamsAs1DForOutWhenUnconnected=off
  wires:
  divide by delta T/1 -> dy(t)/dt/1
  Delay1/1 -> Sum6/1
  "if we went through a \"step\""/1 -> Hold this value/Action
  Hold this value/1(Out1) -> divide by delta T/1
  Sum6/1 -> "if we went through a \"step\""/1, Hold this value/1(In1)
  y(t)/1 -> Sum6/2, Delay1/2, Delay1/1

== system CLVF/Phase #3: Experiment/Change RED Behavior/Sub-Phase #1/Custom Discrete PD (Y-Position)/x_dot -> x1 ==
  note: dy/dt ~= (y2-y1)/deltaT
  y(t) : Inport
  Delay1 : Delay  DelayLength=1  InitialConditionSource=Input port
      settings: InputPortMap=u0,p4
  Hold this value : Subsystem  TreatAsAtomicUnit=on
  Sum6 : Sum  Inputs=-+|
  divide by delta T : Gain  Gain=1/serverRate
  "if we went through a \"step\"" : If  IfExpression=u1 ~= 0  ShowElse=off
  dy(t)/dt : Outport  VectorParamsAs1DForOutWhenUnconnected=off
  wires:
  divide by delta T/1 -> dy(t)/dt/1
  Delay1/1 -> Sum6/1
  "if we went through a \"step\""/1 -> Hold this value/Action
  Hold this value/1(Out1) -> divide by delta T/1
  Sum6/1 -> "if we went through a \"step\""/1, Hold this value/1(In1)
  y(t)/1 -> Sum6/2, Delay1/2, Delay1/1

== system CLVF/Phase #3: Experiment/Change RED Behavior/Sub-Phase #4/Custom Discrete PD (Attitude)/x_dot -> x1 ==
  note: dy/dt ~= (y2-y1)/deltaT
  y(t) : Inport
  Delay1 : Delay  DelayLength=1  InitialConditionSource=Input port
      settings: InputPortMap=u0,p4
  Hold this value : Subsystem  TreatAsAtomicUnit=on
  Sum6 : Sum  Inputs=-+|
  divide by delta T : Gain  Gain=1/serverRate
  "if we went through a \"step\"" : If  IfExpression=u1 ~= 0  ShowElse=off
  dy(t)/dt : Outport  VectorParamsAs1DForOutWhenUnconnected=off
  wires:
  divide by delta T/1 -> dy(t)/dt/1
  Delay1/1 -> Sum6/1
  "if we went through a \"step\""/1 -> Hold this value/Action
  Hold this value/1(Out1) -> divide by delta T/1
  Sum6/1 -> "if we went through a \"step\""/1, Hold this value/1(In1)
  y(t)/1 -> Sum6/2, Delay1/2, Delay1/1

== system CLVF/Phase #3: Experiment/Change RED Behavior/Sub-Phase #4/Custom Discrete PD (X-Position)/x_dot -> x1 ==
  note: dy/dt ~= (y2-y1)/deltaT
  y(t) : Inport
  Delay1 : Delay  DelayLength=1  InitialConditionSource=Input port
      settings: InputPortMap=u0,p4
  Hold this value : Subsystem  TreatAsAtomicUnit=on
  Sum6 : Sum  Inputs=-+|
  divide by delta T : Gain  Gain=1/serverRate
  "if we went through a \"step\"" : If  IfExpression=u1 ~= 0  ShowElse=off
  dy(t)/dt : Outport  VectorParamsAs1DForOutWhenUnconnected=off
  wires:
  divide by delta T/1 -> dy(t)/dt/1
  Delay1/1 -> Sum6/1
  "if we went through a \"step\""/1 -> Hold this value/Action
  Hold this value/1(Out1) -> divide by delta T/1
  Sum6/1 -> "if we went through a \"step\""/1, Hold this value/1(In1)
  y(t)/1 -> Sum6/2, Delay1/2, Delay1/1

== system CLVF/Phase #3: Experiment/Change RED Behavior/Sub-Phase #4/Custom Discrete PD (Y-Position)/x_dot -> x1 ==
  note: dy/dt ~= (y2-y1)/deltaT
  y(t) : Inport
  Delay1 : Delay  DelayLength=1  InitialConditionSource=Input port
      settings: InputPortMap=u0,p4
  Hold this value : Subsystem  TreatAsAtomicUnit=on
  Sum6 : Sum  Inputs=-+|
  divide by delta T : Gain  Gain=1/serverRate
  "if we went through a \"step\"" : If  IfExpression=u1 ~= 0  ShowElse=off
  dy(t)/dt : Outport  VectorParamsAs1DForOutWhenUnconnected=off
  wires:
  divide by delta T/1 -> dy(t)/dt/1
  Delay1/1 -> Sum6/1
  "if we went through a \"step\""/1 -> Hold this value/Action
  Hold this value/1(Out1) -> divide by delta T/1
  Sum6/1 -> "if we went through a \"step\""/1, Hold this value/1(In1)
  y(t)/1 -> Sum6/2, Delay1/2, Delay1/1

== system CLVF/Phase #4: Return Home/Change BLACK Behavior/Custom Discrete PD (Attitude)/x_dot -> x1/Hold this value ==
  In1 : Inport
  Action Port : ActionPort  ActionPortLabel=if(u1 ~= 0)
  Out1 : Outport  VectorParamsAs1DForOutWhenUnconnected=off
  wires:
  In1/1 -> Out1/1

== system CLVF/Phase #4: Return Home/Change BLACK Behavior/Custom Discrete PD (X-Position)/x_dot -> x1/Hold this value ==
  In1 : Inport
  Action Port : ActionPort  ActionPortLabel=if(u1 ~= 0)
  Out1 : Outport  VectorParamsAs1DForOutWhenUnconnected=off
  wires:
  In1/1 -> Out1/1

== system CLVF/Phase #4: Return Home/Change BLACK Behavior/Custom Discrete PD (Y-Position)/x_dot -> x1/Hold this value ==
  In1 : Inport
  Action Port : ActionPort  ActionPortLabel=if(u1 ~= 0)
  Out1 : Outport  VectorParamsAs1DForOutWhenUnconnected=off
  wires:
  In1/1 -> Out1/1

== system CLVF/Phase #4: Return Home/Change BLUE Behavior/Custom Discrete PD (Attitude)/x_dot -> x1/Hold this value ==
  In1 : Inport
  Action Port : ActionPort  ActionPortLabel=if(u1 ~= 0)
  Out1 : Outport  VectorParamsAs1DForOutWhenUnconnected=off
  wires:
  In1/1 -> Out1/1

== system CLVF/Phase #4: Return Home/Change BLUE Behavior/Custom Discrete PD (X-Position)/x_dot -> x1/Hold this value ==
  In1 : Inport
  Action Port : ActionPort  ActionPortLabel=if(u1 ~= 0)
  Out1 : Outport  VectorParamsAs1DForOutWhenUnconnected=off
  wires:
  In1/1 -> Out1/1

== system CLVF/Phase #4: Return Home/Change BLUE Behavior/Custom Discrete PD (Y-Position)/x_dot -> x1/Hold this value ==
  In1 : Inport
  Action Port : ActionPort  ActionPortLabel=if(u1 ~= 0)
  Out1 : Outport  VectorParamsAs1DForOutWhenUnconnected=off
  wires:
  In1/1 -> Out1/1

== system CLVF/Phase #4: Return Home/Change RED Behavior/Custom Discrete PD (Attitude)/x_dot -> x1/Hold this value ==
  In1 : Inport
  Action Port : ActionPort  ActionPortLabel=if(u1 ~= 0)
  Out1 : Outport  VectorParamsAs1DForOutWhenUnconnected=off
  wires:
  In1/1 -> Out1/1

== system CLVF/Phase #4: Return Home/Change RED Behavior/Custom Discrete PD (X-Position)/x_dot -> x1/Hold this value ==
  In1 : Inport
  Action Port : ActionPort  ActionPortLabel=if(u1 ~= 0)
  Out1 : Outport  VectorParamsAs1DForOutWhenUnconnected=off
  wires:
  In1/1 -> Out1/1

== system CLVF/Phase #4: Return Home/Change RED Behavior/Custom Discrete PD (Y-Position)/x_dot -> x1/Hold this value ==
  In1 : Inport
  Action Port : ActionPort  ActionPortLabel=if(u1 ~= 0)
  Out1 : Outport  VectorParamsAs1DForOutWhenUnconnected=off
  wires:
  In1/1 -> Out1/1

== system CLVF/Phase #5: Hold Home/Change BLACK Behavior/Custom Discrete PD (Attitude)/x_dot -> x1/Hold this value ==
  In1 : Inport
  Action Port : ActionPort  ActionPortLabel=if(u1 ~= 0)
  Out1 : Outport  VectorParamsAs1DForOutWhenUnconnected=off
  wires:
  In1/1 -> Out1/1

== system CLVF/Phase #5: Hold Home/Change BLACK Behavior/Custom Discrete PD (X-Position)/x_dot -> x1/Hold this value ==
  In1 : Inport
  Action Port : ActionPort  ActionPortLabel=if(u1 ~= 0)
  Out1 : Outport  VectorParamsAs1DForOutWhenUnconnected=off
  wires:
  In1/1 -> Out1/1

== system CLVF/Phase #5: Hold Home/Change BLACK Behavior/Custom Discrete PD (Y-Position)/x_dot -> x1/Hold this value ==
  In1 : Inport
  Action Port : ActionPort  ActionPortLabel=if(u1 ~= 0)
  Out1 : Outport  VectorParamsAs1DForOutWhenUnconnected=off
  wires:
  In1/1 -> Out1/1

== system CLVF/Phase #5: Hold Home/Change BLUE Behavior/Custom Discrete PD (Attitude)/x_dot -> x1/Hold this value ==
  In1 : Inport
  Action Port : ActionPort  ActionPortLabel=if(u1 ~= 0)
  Out1 : Outport  VectorParamsAs1DForOutWhenUnconnected=off
  wires:
  In1/1 -> Out1/1

== system CLVF/Phase #5: Hold Home/Change BLUE Behavior/Custom Discrete PD (X-Position)/x_dot -> x1/Hold this value ==
  In1 : Inport
  Action Port : ActionPort  ActionPortLabel=if(u1 ~= 0)
  Out1 : Outport  VectorParamsAs1DForOutWhenUnconnected=off
  wires:
  In1/1 -> Out1/1

== system CLVF/Phase #5: Hold Home/Change BLUE Behavior/Custom Discrete PD (Y-Position)/x_dot -> x1/Hold this value ==
  In1 : Inport
  Action Port : ActionPort  ActionPortLabel=if(u1 ~= 0)
  Out1 : Outport  VectorParamsAs1DForOutWhenUnconnected=off
  wires:
  In1/1 -> Out1/1

== system CLVF/Phase #5: Hold Home/Change RED Behavior/Custom Discrete PD (Attitude)/x_dot -> x1/Hold this value ==
  In1 : Inport
  Action Port : ActionPort  ActionPortLabel=if(u1 ~= 0)
  Out1 : Outport  VectorParamsAs1DForOutWhenUnconnected=off
  wires:
  In1/1 -> Out1/1

== system CLVF/Phase #5: Hold Home/Change RED Behavior/Custom Discrete PD (X-Position)/x_dot -> x1/Hold this value ==
  In1 : Inport
  Action Port : ActionPort  ActionPortLabel=if(u1 ~= 0)
  Out1 : Outport  VectorParamsAs1DForOutWhenUnconnected=off
  wires:
  In1/1 -> Out1/1

== system CLVF/Phase #5: Hold Home/Change RED Behavior/Custom Discrete PD (Y-Position)/x_dot -> x1/Hold this value ==
  In1 : Inport
  Action Port : ActionPort  ActionPortLabel=if(u1 ~= 0)
  Out1 : Outport  VectorParamsAs1DForOutWhenUnconnected=off
  wires:
  In1/1 -> Out1/1

== system CLVF/Grab PhaseSpace Data via UDP/Use Hardware to Obtain States/Using RED+BLACK, or RED+BLACK+ARM/Obtain BLACK States/x_dot -> x1/Hold this value ==
  In1 : Inport
  Action Port : ActionPort
  Out1 : Outport  VectorParamsAs1DForOutWhenUnconnected=off
  wires:
  In1/1 -> Out1/1

== system CLVF/Grab PhaseSpace Data via UDP/Use Hardware to Obtain States/Using RED+BLACK, or RED+BLACK+ARM/Obtain BLACK States/x_dot -> x10/Hold this value ==
  In1 : Inport
  Action Port : ActionPort
  Out1 : Outport  VectorParamsAs1DForOutWhenUnconnected=off
  wires:
  In1/1 -> Out1/1
